simulink model "ai_dr_screening"
settings: Solver=VariableStepAuto  StartTime=0.0  StopTime=28800.0
undefined symbols (not defined in the file or in its folder): simParams
Description:
  | Complete dynamic simulation model of rural Indian diabetic retinopathy screening: Patient Arrival -> Fundus Camera Acquisition -> Network Uplink Delay -> IQA Usable Check & Recapture -> Automated AI (EfficientNet + U-Net + Grad-CAM + SHAP) -> Referral Engine -> Human Ophthalmologist Review Pool.
settings Model: Creator=AI DR Screen — Retina Rovers  LastModifiedBy=Mithres P

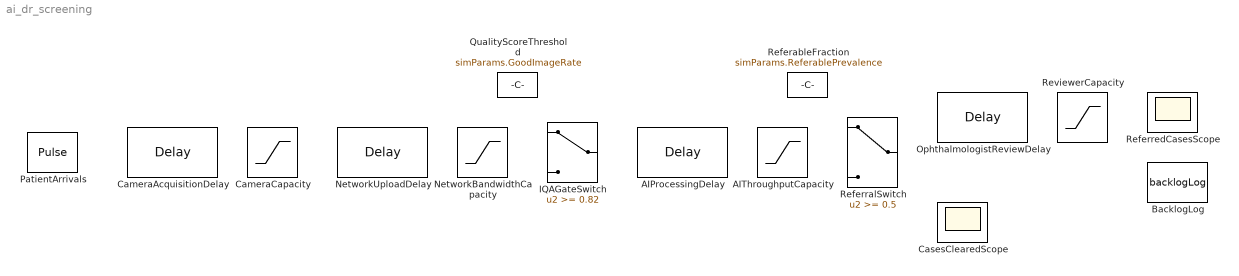
== system ai_dr_screening ==
  PatientArrivals : PulseGenerator  Period=3600/simParams.PatientArrivalRatePerHour  PulseWidth=10  Amplitude=1
  CameraAcquisitionDelay : TransportDelay  DelayTime=simParams.AcquisitionSecPerImage
  CameraCapacity : Saturate  UpperLimit=simParams.CameraCount  LowerLimit=0
  NetworkUploadDelay : TransportDelay  DelayTime=simParams.UploadTimePerImageSec
  NetworkBandwidthCapacity : Saturate  UpperLimit=max(1, ceil(simParams.BandwidthMbps/2.0))  LowerLimit=0
  IQAGateSwitch : Switch  Criteria=u2 >= Threshold  Threshold=0.82
  QualityScoreThreshold : Constant  Value=simParams.GoodImageRate
  AIProcessingDelay : TransportDelay  DelayTime=simParams.TotalAIProcessingSec
  AIThroughputCapacity : Saturate  UpperLimit=simParams.AIWorkerInstances  LowerLimit=0
  ReferralSwitch : Switch  Criteria=u2 >= Threshold  Threshold=0.5
  ReferableFraction : Constant  Value=simParams.ReferablePrevalence
  OphthalmologistReviewDelay : TransportDelay  DelayTime=simParams.ReviewSecPerCase
  ReviewerCapacity : Saturate  UpperLimit=simParams.OphthalmologistCount  LowerLimit=0
  CasesClearedScope : Scope
  ReferredCasesScope : Scope
  BacklogLog : ToWorkspace  VariableName=backlogLog  SaveFormat=Timeseries
  wires:
  ?PatientArrivals/1 -> ?CameraAcquisitionDelay/1
  ?CameraAcquisitionDelay/1 -> ?CameraCapacity/1
  ?CameraCapacity/1 -> ?NetworkUploadDelay/1
  ?NetworkUploadDelay/1 -> ?NetworkBandwidthCapacity/1
  ?NetworkBandwidthCapacity/1 -> ?IQAGateSwitch/2
  ?QualityScoreThreshold/1 -> ?IQAGateSwitch/1
  ?IQAGateSwitch/1 -> ?AIProcessingDelay/1
  ?AIProcessingDelay/1 -> ?AIThroughputCapacity/1
  ?AIThroughputCapacity/1 -> ?ReferralSwitch/2
  ?ReferableFraction/1 -> ?ReferralSwitch/1
  ?ReferralSwitch/1 -> ?OphthalmologistReviewDelay/1
  ?ReferralSwitch/2 -> ?CasesClearedScope/1
  ?OphthalmologistReviewDelay/1 -> ?ReviewerCapacity/1
  ?ReviewerCapacity/1 -> ?ReferredCasesScope/1
  ?ReviewerCapacity/1 -> ?BacklogLog/1
